simulink model "SolarPVMPPTBoost"  (R2025a)
settings: Solver=ode23t  StartTime=0.0  StopTime=simulation.timeSim  MaxStep=1/(10*solarPlant.converterSwitchingFrequency)  RelTol=1e-3  AbsTol=1e-3
PreLoadFcn:
  | run('SolarPVMPPTBoostData');
undefined symbols (not defined in the file or in its folder): boostController, dcVoltage, sensor, solarPanel, solarPlant
libraries: fl_lib x13, nesl_utility x9, simulink x6, ee_lib x3, eePwmGenerator x2, simulink_extras x1
Description:
  | Solar PV System with MPPT Using Boost Converter
  | 
  | %
settings Model: Creator=The MathWorks, Inc.  LastModifiedBy=The MathWorks, Inc.
settings SolverCC: AutoScaleAbsTol=off  AlgebraicLoopSolver=TrustRegion  MaxZcPerStep=1.0
settings DataIOCC: SaveOutput=off  DSMLogging=off  SaveTime=off  ReturnWorkspaceOutputs=off  SignalLoggingName=SolarPVMPPTBoost_logDB
settings OptimizationCC: ReuseModelBlockBuffer=off
settings DebuggingCC: UnconnectedInputMsg=warning  UnconnectedOutputMsg=warning  UnconnectedLineMsg=warning  SymbolicDimsDataTypeCodeGenerationDiagnostic=none
settings ModelReferenceCC: EnableRefExpFcnMdlSchedulingChecks=on
settings SFSimCC: CustomCodeUndefinedFunction=UseInterfaceOnly
settings RTWCC: GPUComputeCapability=3.5  DLArmComputeVersion=19.05
settings SimscapeCC: SimscapeLogType=all  SimscapeLogSimulationStatistics=on  SimscapeLogName=simlog_SolarPVMPPTBoost  SimscapeLogDataHistory=10000.0

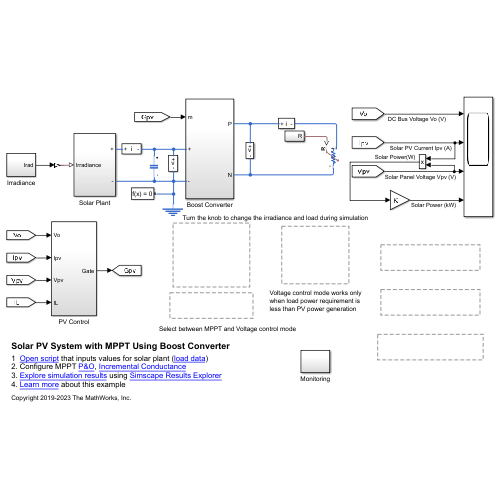
[thumbnail: Simulink's stored preview of the top-level diagram]
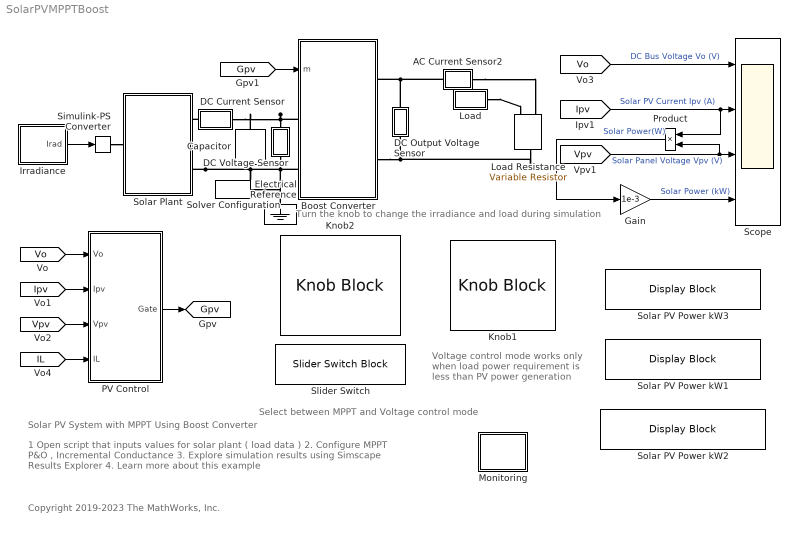
== system SolarPVMPPTBoost ==
  note: Turn the knob to change the irradiance and load during simulation
  note: Select between MPPT and Voltage control mode
  note: Voltage control mode works only when load power requirement is less than PV power generation
  note: Solar PV System with MPPT Using Boost Converter
  note: 1 Open script that inputs values for solar plant ( load data )
      | 2. Configure MPPT P&O , Incremental Conductance
      | 3. Explore simulation results using Simscape Results Explorer
      | 4. Learn more about this example
  note: Copyright 2019-2023 The MathWorks, Inc.
  AC Current Sensor2 : Subsystem
      mask Display: disp('i');
  Boost Converter : Subsystem  VariantControl=boostCircuit == 1
  Capacitor : fl_lib/Electrical/Electrical Elements/Capacitor  c=boost.inputCapacitor F  r=1e-6 Ohm  g=0 1/Ohm  i_specify=off  i_priority=None  i=0 A  i_nominal_specify=off  i_nominal_value=1  i_nominal_unit=A  v_specify=off  v_priority=None  v=solarPlant.startMPPTValue V  v_nominal_specify=off  v_nominal_value=1  v_nominal_unit=V  vc_specify=on  vc_priority=High  vc=solarPlant.startMPPTValue V  vc_nominal_specify=off  vc_nominal_value=1  vc_nominal_unit=V
  DC Current Sensor : Subsystem
      mask Display: disp('i')
  DC Output Voltage Sensor : Subsystem
      mask Display: disp('v')
  DC Voltage Sensor : Subsystem
      mask Display: disp('v');
  Electrical Reference : fl_lib/Electrical/Electrical Elements/Electrical Reference
  Gain : Gain  Gain=1e-3
  Irradiance : Subsystem
  Knob1 : KnobBlock  ScaleMin=0.1  ScaleMax=2  TickInterval=0.2
  Knob2 : KnobBlock  ScaleMin=150  ScaleMax=1000
  Load : Subsystem
  Load Resistance : fl_lib/Electrical/Electrical Elements/Variable Resistor  Rmin=0 Ohm  thermalEnable=false  thermal_mass=1 J/K  i_specify=off  i_priority=None  i=5 A  i_nominal_specify=off  i_nominal_value=1  i_nominal_unit=A  v_specify=off  v_priority=None  v=0 V  v_nominal_specify=off  v_nominal_value=1  v_nominal_unit=V  T_specify=off  T_priority=None  T=300 K  T_nominal_specify=off  T_nominal_value=1  T_nominal_unit=K
  Monitoring : Subsystem
  PV Control : Subsystem
  Product : Product
  Scope : Scope  NumInputPorts=4
      settings: TimeSpan=simulation.timeSim  ActiveDisplayYMinimum=-66.02811  ActiveDisplayYMaximum=594.25302
  Simulink-PS Converter : nesl_utility/Simulink-PS Converter  PhysicalDomain=network_engine_domain  SubClassName=ps_input  LeftPortType=input  RightPortType=output  PseudoPeriodic=off  Frequencies=[]  NoiseDistribution=none  NoiseParameters=[]  Unit=1  AffineConversion=off  FilteringAndDerivatives=provide  SimscapeFilterOrder=1  InputFilterTimeConstant=0.001  UdotUserProvided=0
  Slider Switch : SliderSwitchBlock
  Solar PV Power kW1 : DisplayBlock  Transparency=1  GridColor=[0.502, 0.502, 0.502]
  Solar PV Power kW2 : DisplayBlock  Transparency=1  GridColor=[0.502, 0.502, 0.502]
  Solar PV Power kW3 : DisplayBlock  Transparency=1  GridColor=[0.502, 0.502, 0.502]
  Solar Plant : Subsystem
  Solver Configuration : nesl_utility/Solver Configuration  PhysicalDomain=network_engine_domain  SubClassName=solver  LeftPortType=input  RightPortType=generic  Tones=[]  Harmonics=[]  SimulateNoise=off  Profile=off  UseLocalSampling=off  EnableSwitchedLinearOptims=on  FrequencyDomain=off  UseCCode=off  RelTol=0.001  AbsTol=1e-06  MinStep=1e-09  ToWorkspace=off  RevertToSquareIcSolve=off  NumHomotopyIterations=100  PhasorMode=off  PhasorModeNumHarmonics=1  ConsistencySolver=NEWTON_FTOL  IndexReductionMethod=DerivativeReplacement  DoDC=off  ResidualTolerance=1e-9  ConsistencyTolSource=GLOBAL  ConsistencyAbsTol=0.001  ConsistencyRelTol=0.001  ConsistencyTolFactor=0.001  UseLocalSolver=off  LocalSolverChoice=NE_BACKWARD_EULER_ADVANCER  ResolveIndetEquations=on  FunctionEvalNumThread=1  LocalSolverSampleTime=1e-6  DoFixedCost=off  MaxNonlinIter=10  MaxModeIter=2  ComputeImpulses=off  ImpulseIterations=2  LinearAlgebra=auto  LinearAlgebraNumThread=0  EquationFormulation=NE_TIME_EF  DelaysMemoryBudget=1024  AutomaticFiltering=on  FilteringTimeConstant=0.001  PartitionStorageMethod=AS_NEEDED  PartitionMemoryBudget=1024  PartitionMethod=FAST  MultibodyUseLocalSolver=off  MultibodyLocalSolverChoice=ODE1  MultibodyLocalSolverSampleTime=0.001
  tag scope: Gpv=global
  wires:
  PV Control/1(Gate) -> [Gpv]
  [Vo] -> Scope/1  "DC Bus Voltage Vo (V)"
  Irradiance/1(Irad) -> Simulink-PS Converter/1
  [Vpv] -> Product/2, Scope/3  "Solar Panel Voltage Vpv (V)"
  [Gpv] -> Boost Converter/1(m)
  [Vo] -> PV Control/1(Vo)
  [Ipv] -> Product/1, Scope/2  "Solar PV Current Ipv (A)"
  Product/1 -> Gain/1  "Solar Power(W)"
  Gain/1 -> Scope/4  "Solar Power (kW)"
  [Ipv] -> PV Control/2(Ipv)
  [Vpv] -> PV Control/3(Vpv)
  [IL] -> PV Control/4(IL)
  connections:
  Boost Converter/RConn2 -- Load Resistance/RConn1 -- DC Output Voltage Sensor/LConn1
  Solar Plant/RConn2 -- Solver Configuration/RConn1 -- Electrical Reference/LConn1 -- Boost Converter/LConn2 -- DC Voltage Sensor/LConn1 -- Capacitor/RConn1
  DC Voltage Sensor/RConn1 -- DC Current Sensor/LConn1 -- Capacitor/LConn1 -- Boost Converter/LConn1
  DC Output Voltage Sensor/RConn1 -- AC Current Sensor2/RConn1 -- Boost Converter/RConn1
  Simulink-PS Converter/RConn1 -- Solar Plant/LConn1
  DC Current Sensor/RConn1 -- Solar Plant/RConn1
  Load/RConn1 -- Load Resistance/LConn1
  AC Current Sensor2/LConn1 -- Load Resistance/LConn2

== system SolarPVMPPTBoost/AC Current Sensor2 ==
  Current Sensor : fl_lib/Electrical/Electrical Sensors/Current Sensor
  PS-Simulink Converter : nesl_utility/PS-Simulink Converter  PhysicalDomain=network_engine_domain  SubClassName=ps_output  LeftPortType=input  RightPortType=output  PseudoPeriodic=off  Frequencies=[]  VectorFormat=1-D array  Unit=1  AffineConversion=off
  Sensor dynamics : TransferFcn  Numerator=1  Denominator=[1/sensor.samplingFreq 1]
  - : PMIOPort  Side=Left
  + : PMIOPort  Port=2  Side=Right
  tag scope: Iload=global
  wires:
  PS-Simulink Converter/1 -> Sensor dynamics/1
  Sensor dynamics/1 -> [Iload]
  connections:
  Current Sensor/RConn1 -- PS-Simulink Converter/LConn1
  +/RConn1 -- Current Sensor/LConn1
  Current Sensor/RConn2 -- -/RConn1

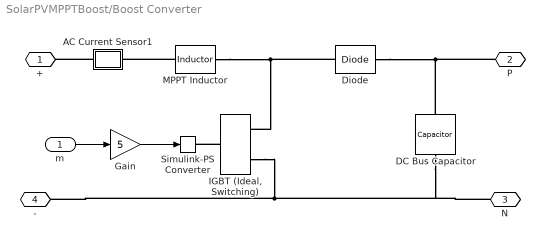
== system SolarPVMPPTBoost/Boost Converter ==
  m : Inport
  AC Current Sensor1 : Subsystem
      mask Display: disp('i');
  DC Bus Capacitor : fl_lib/Electrical/Electrical Elements/Capacitor  c=boost.outputCapacitor F  r=1e-6 Ohm  g=0 1/Ohm  i_specify=off  i_priority=None  i=0 A  i_nominal_specify=off  i_nominal_value=1  i_nominal_unit=A  v_specify=off  v_priority=None  v=0 V  v_nominal_specify=off  v_nominal_value=1  v_nominal_unit=V  vc_specify=on  vc_priority=High  vc=dcVoltage.avgDCVoltage V  vc_nominal_specify=off  vc_nominal_value=1  vc_nominal_unit=V
  Diode : fl_lib/Electrical/Electrical Elements/Diode  Vf=0.6 V  Ron=0.3 Ohm  Goff=1e-8 1/Ohm  i_specify=off  i_priority=None  i=0 A  i_nominal_specify=off  i_nominal_value=1  i_nominal_unit=A  v_specify=off  v_priority=None  v=0 V  v_nominal_specify=off  v_nominal_value=1  v_nominal_unit=V
  Gain : Gain  Gain=5
  "IGBT (Ideal, Switching)" : ee_lib/Semiconductors & Converters/IGBT (Ideal, Switching)  port_option=ee.enum.controlport.ps  Vf=0.8 V  Ron=0.001 Ohm  Goff=1e-5 1/Ohm  Vth=2.5 V  diode_param=1  diode_Vf=0.8 V  diode_Ron=0.001 Ohm  diode_Goff=1e-5 1/Ohm  diode_C=50e-9 F  diode_iRM=-235 A  diode_iF=300 A  diode_idot=-50 A/us  diode_trr_param=1  diode_trr_factor=3  diode_trr=15 us  diode_Qrr=1500 s*uA  ice_specify=off  ice_priority=None  ice=0 A  ice_nominal_specify=off  ice_nominal_value=1  ice_nominal_unit=A  vce_specify=off  vce_priority=None  vce=0 V  vce_nominal_specify=off  vce_nominal_value=1  vce_nominal_unit=V  vge_specify=off  vge_priority=None  vge=0 V  vge_nominal_specify=off  vge_nominal_value=1  vge_nominal_unit=V  thermal_loss_option=ee.enum.converters.thermalLossOption.constantvalues  Von_data=[0, .1, .6, .8, 1, 1.3, 1.6, 2, 2.4; 0, .1, .7, 1, 1.2, 1.5, 1.9, 2.4, 2.8] V  Tj=[298.15, 398.15] K  Iout_data=[0, .1, 1, 5, 10, 20, 40, 70, 100] A  Eon_data=[0, .0024, .024, .12, .2, .48, 1.04, 2.16, 3.24; 0, .003, .03, .15, .25, .6, 1.3, 2.7, 4.05] * 1e-3 J  Eoff_data=[0, .0007, .0066, .033, .066, .17, .33, .83, 1.5; 0, .001, .01, .05, .1, .25, .5, 1.2, 2.2] * 1e-3 J  Eon_data_3D=[zeros(2, 9, 3)] J  Eoff_data_3D=[zeros(2, 9, 3)] J  Tj_loss=[298.15, 398.15] K  Iout_data_loss=[0, .1, 1, 5, 10, 20, 40, 70, 100] A  tabulateWithVce=false  Vce_loss=[0, 150, 300] V  Eon_scalar=22.86e-3 J  Eoff_scalar=17.14e-3 J  Voff=300 V  Iout_scalar=600 A  useCurrentFromPreviousCycle=false  useVoltageFromPreviousCycle=false  diodeModelType=ee.enum.converters.diodeModelType.pwl  diodeTableType=ee.enum.diode.tableType.IfMat  diode_ReverseIVType=ee.enum.diode.diodeReverseIV.constant  diode_IfMat=[.07, .12, .19, 1.75, 4.24, 7.32, 11.2; .16, .3, .72, 2.14, 4.02, 6.35, 9.12] A  diode_VfMat=[.9, 1.15, 1.25, 1.5, 1.75, 2.17, 2.6, 2.85; .58, .68, .75, 1.1, 1.38, 1.77, 2.27, 2.7] V  diode_TjVec=[25, 125] degC  diode_VfVec=[.5, .7, .9, 1.3, 1.7, 2.1, 2.5] V  diode_IfVec=[.1, .2, .5, 1, 2, 4, 7, 10] A  diode_IrMat=[1e-06, 2e-06, 5e-06, 1e-05, 2.5e-05, 5e-05, .0001; 2e-06, 5e-06, 1e-05, 4e-05, 8e-05, .0002, .0005] A  diode_VrMat=[10, 100, 200, 250, 300, 325, 350; 10, 70, 160, 220, 270, 300, 320] V  diode_VrVec=[10, 20, 40, 50, 70, 80, 100] V  diode_IrVec=[1e-06, 2e-06, 5e-06, 1e-05, 2e-05, 5e-05, .0001] A  diode_Vr=-600 V  diode_Ls=150 nH  diode_Erec=0.03 J  diode_rec_loss_model=ee.enum.diode.reverseRecoveryModel.fixed  diode_ErecVal=0 J  diode_scaleWithIandV=true  diode_ErecMat=zeros(2, 3) J  diode_TjrecVec=[298.15, 398.15] K  diode_IfrecVec=[.1, 1, 10] A  diode_IrecVal=10 A  diode_VrecVal=10 V  diode_tFilter=1 / 1000 / 100 s  separateThermalPortForDiode=false  thermal_network_parameterization=ee.enum.thermalNetworkTopology.external  Rth=[.08, .5] K/W  Rth_Cauer=[.08, .1, .5] K/W  Rth_Foster=[.08, .14, .22, .16] K/W  thermal_mass_parameterization=ee.enum.thermalNetwork.timeconstant  thermal_mass=[.01, .5] J/K  thermal_mass_Cauer=[.01, .1, .5] J/K  thermal_mass_Foster=[.001, .005, .05, .5] J/K  thermal_time_constant=[.001, .2] s  thermal_time_constant_Cauer=[.001, .1, .2] s  thermal_time_constant_Foster=[7e-05, .0007, .01, .08] s  thermal_mass_initial_temperatures=[25, 25] degC  thermal_mass_initial_temperatures_Cauer=[25, 25, 25] degC  junction_thermal_mass=0.01 J/K  Tvec_initial_Foster=[25, 25, 25, 25] degC  RthDiode=[.03, .2] K/W  RthCauerDiode=[.03, .1, .2] K/W  RthFosterDiode=[.03, .2] K/W  thermalMassDiode=[3, 25] J/K  thermalMassCauerDiode=[3, 10, 25] J/K  thermalMassFosterDiode=[33, 50] J/K  thermalTauDiode=[.1, 5] s  thermalTauCauerDiode=[.1, 1, 5] s  thermalTauFosterDiode=[1, 10] s  thermalMassInitTempDiode=[25, 25] degC  thermalMassInitTempCauerDiode=[25, 25, 25] degC  junctionthermalMassDiode=0.1 J/K  TVecInitialFosterDiode=[25, 25, 25, 25] degC  no_thermal_network=0  IGBT_junction_temperature_specify=off  IGBT_junction_temperature_priority=None  IGBT_junction_temperature=25 degC  IGBT_junction_temperature_nominal_specify=off  IGBT_junction_temperature_nominal_value=1  IGBT_junction_temperature_nominal_unit=degC  diode_junction_temperature_specify=off  diode_junction_temperature_priority=None  diode_junction_temperature=25 degC  diode_junction_temperature_nominal_specify=off  diode_junction_temperature_nominal_value=1  diode_junction_temperature_nominal_unit=degC  Qj_specify=off  Qj_priority=None  Qj=0 W  Qj_nominal_specify=off  Qj_nominal_value=1  Qj_nominal_unit=W  accumulatedSwitchingLosses_specify=off  accumulatedSwitchingLosses_priority=None  accumulatedSwitchingLosses=0 J
  MPPT Inductor : ee_lib/Passive/Inductor  l=boost.inductor H  enable_L_tol=0  L_tol=5  tol_distribution=1  nSigma=4  r=boost.inductorResistance Ohm  g=1e-9 1/Ohm  enable_operating_limits=0  operating_limit_action=2  max_working_current=1 A  power_rating=1 W  i_L_specify=on  i_L_priority=High  i_L=0 A  i_L_nominal_specify=off  i_L_nominal_value=1  i_L_nominal_unit=A
  Simulink-PS Converter : nesl_utility/Simulink-PS Converter  PhysicalDomain=network_engine_domain  SubClassName=ps_input  LeftPortType=input  RightPortType=output  PseudoPeriodic=off  Frequencies=[]  NoiseDistribution=none  NoiseParameters=[]  Unit=1  AffineConversion=off  FilteringAndDerivatives=provide  SimscapeFilterOrder=1  InputFilterTimeConstant=0.001  UdotUserProvided=0
  + : PMIOPort  Side=Left
  P : PMIOPort  Port=2  Side=Right
  N : PMIOPort  Port=3  Side=Right
  - : PMIOPort  Port=4  Side=Left
  wires:
  m/1 -> Gain/1
  Gain/1 -> Simulink-PS Converter/1
  connections:
  MPPT Inductor/LConn1 -- AC Current Sensor1/LConn1
  "IGBT (Ideal, Switching)"/RConn2 -- N/RConn1 -- DC Bus Capacitor/RConn1 -- -/RConn1
  AC Current Sensor1/RConn1 -- +/RConn1
  "IGBT (Ideal, Switching)"/LConn1 -- Simulink-PS Converter/RConn1
  MPPT Inductor/RConn1 -- "IGBT (Ideal, Switching)"/RConn1 -- Diode/LConn1
  DC Bus Capacitor/LConn1 -- Diode/RConn1 -- P/RConn1

== system SolarPVMPPTBoost/DC Current Sensor ==
  Current Sensor : fl_lib/Electrical/Electrical Sensors/Current Sensor
      settings: LogSimulationData=on
  PS-Simulink Converter : nesl_utility/PS-Simulink Converter  PhysicalDomain=network_engine_domain  SubClassName=ps_output  LeftPortType=input  RightPortType=output  PseudoPeriodic=off  Frequencies=[]  VectorFormat=1-D array  Unit=1  AffineConversion=off
  Sensor dynamics : TransferFcn  Numerator=1  Denominator=[1/sensor.samplingFreq 1]
  - : PMIOPort  Side=Left
  + : PMIOPort  Port=2  Side=Right
  tag scope: Ipv=global
  wires:
  PS-Simulink Converter/1 -> Sensor dynamics/1
  Sensor dynamics/1 -> [Ipv]
  connections:
  Current Sensor/RConn2 -- -/RConn1
  +/RConn1 -- Current Sensor/LConn1
  Current Sensor/RConn1 -- PS-Simulink Converter/LConn1

== system SolarPVMPPTBoost/DC Output Voltage Sensor ==
  PS-Simulink Converter : nesl_utility/PS-Simulink Converter  PhysicalDomain=network_engine_domain  SubClassName=ps_output  LeftPortType=input  RightPortType=output  PseudoPeriodic=off  Frequencies=[]  VectorFormat=1-D array  Unit=1  AffineConversion=off
  Sensor dynamics : TransferFcn  Numerator=1  Denominator=[1/sensor.samplingFreq 1]
  Voltage Sensor : fl_lib/Electrical/Electrical Sensors/Voltage Sensor
  - : PMIOPort  Side=Left
  + : PMIOPort  Port=2  Side=Right
  tag scope: Vo=global
  wires:
  PS-Simulink Converter/1 -> Sensor dynamics/1
  Sensor dynamics/1 -> [Vo]
  connections:
  Voltage Sensor/RConn2 -- -/RConn1
  Voltage Sensor/RConn1 -- PS-Simulink Converter/LConn1
  Voltage Sensor/LConn1 -- +/RConn1

== system SolarPVMPPTBoost/DC Voltage Sensor ==
  PS-Simulink Converter : nesl_utility/PS-Simulink Converter  PhysicalDomain=network_engine_domain  SubClassName=ps_output  LeftPortType=input  RightPortType=output  PseudoPeriodic=off  Frequencies=[]  VectorFormat=1-D array  Unit=1  AffineConversion=off
  Sensor dynamics : TransferFcn  Numerator=1  Denominator=[1/sensor.samplingFreq 1]
  Voltage Sensor : fl_lib/Electrical/Electrical Sensors/Voltage Sensor
      settings: LogSimulationData=on
  - : PMIOPort  Side=Left
  + : PMIOPort  Port=2  Side=Right
  tag scope: Vpv=global
  wires:
  PS-Simulink Converter/1 -> Sensor dynamics/1
  Sensor dynamics/1 -> [Vpv]
  connections:
  Voltage Sensor/LConn1 -- +/RConn1
  Voltage Sensor/RConn1 -- PS-Simulink Converter/LConn1
  Voltage Sensor/RConn2 -- -/RConn1

== system SolarPVMPPTBoost/Irradiance ==
  " " : Constant
  Solar Irradiance W/m2 : Gain  Gain=988.0703074137369
  Irad : Outport
  wires:
  " "/1 -> Solar Irradiance W/m2/1
  Solar Irradiance W/m2/1 -> Irad/1

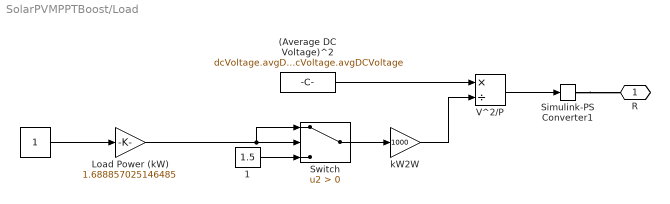
== system SolarPVMPPTBoost/Load ==
  " " : Constant
  " (Average DC Voltage)^2" : Constant  Value=dcVoltage.avgDCVoltage*dcVoltage.avgDCVoltage
  " 1" : Constant  Value=1.5
  Load Power (kW) : Gain  Gain=1.688857025146485
  Simulink-PS Converter1 : nesl_utility/Simulink-PS Converter  PhysicalDomain=network_engine_domain  SubClassName=ps_input  LeftPortType=input  RightPortType=output  PseudoPeriodic=off  Frequencies=[]  NoiseDistribution=none  NoiseParameters=[]  Unit=1  AffineConversion=off  FilteringAndDerivatives=provide  SimscapeFilterOrder=1  InputFilterTimeConstant=0.001  UdotUserProvided=0
  Switch : Switch  Criteria=u2 > Threshold  SaturateOnIntegerOverflow=off  InputSameDT=off
  V^2/P : Product  Inputs=*/
  kW2W : Gain  Gain=1000
  R : PMIOPort  Side=Right
  wires:
  " "/1 -> Load Power (kW)/1
  Load Power (kW)/1 -> Switch/1, Switch/2
  " 1"/1 -> Switch/3
  " (Average DC Voltage)^2"/1 -> V^2/P/1
  V^2/P/1 -> Simulink-PS Converter1/1
  Switch/1 -> kW2W/1
  kW2W/1 -> V^2/P/2
  connections:
  Simulink-PS Converter1/RConn1 -- R/RConn1

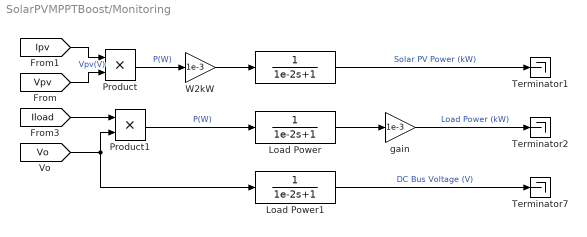
== system SolarPVMPPTBoost/Monitoring ==
  "  " : TransferFcn  Denominator=[1e-2 1]
  Load Power : TransferFcn  Denominator=[1e-2 1]
  Load Power1 : TransferFcn  Denominator=[1e-2 1]
  Product : Product
  Product1 : Product
  Terminator1 : Terminator
  Terminator2 : Terminator
  Terminator7 : Terminator
  W2kW : Gain  Gain=1e-3
  gain : Gain  Gain=1e-3
  wires:
  [Vpv] -> Product/2  "Vpv(V)"
  Load Power/1 -> gain/1
  Product1/1 -> Load Power/1  "P(W)"
  [Iload] -> Product1/1
  "  "/1 -> Terminator1/1  "Solar PV Power (kW)"
  [Ipv] -> Product/1
  [Vo] -> Product1/2, Load Power1/1
  Product/1 -> W2kW/1  "P(W)"
  gain/1 -> Terminator2/1  "Load Power (kW)"
  W2kW/1 -> "  "/1
  Load Power1/1 -> Terminator7/1  "DC Bus Voltage (V)"

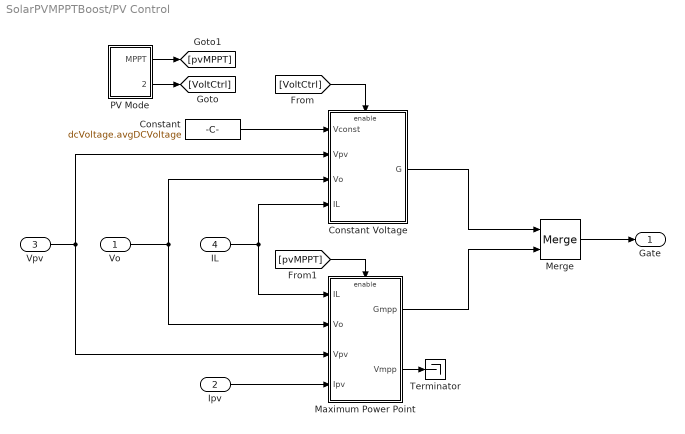
== system SolarPVMPPTBoost/PV Control ==
  Vo : Inport
  Ipv : Inport  Port=2
  Vpv : Inport  Port=3
  IL : Inport  Port=4
  Constant : Constant  Value=dcVoltage.avgDCVoltage
  Constant Voltage : Subsystem
  Maximum Power Point : Subsystem
  Merge : Merge
  PV Mode : Subsystem
  Terminator : Terminator
  Gate : Outport
  wires:
  Merge/1 -> Gate/1
  Vo/1 -> Maximum Power Point/2("Vo "), Constant Voltage/3("Vo ")
  Maximum Power Point/1(Gmpp) -> Merge/2
  [VoltCtrl] -> Constant Voltage/Enable
  IL/1 -> Maximum Power Point/1("IL "), Constant Voltage/4(IL)
  Vpv/1 -> Maximum Power Point/3(Vpv), Constant Voltage/2(Vpv)
  Ipv/1 -> Maximum Power Point/4(Ipv)
  Constant/1 -> Constant Voltage/1(Vconst)
  Constant Voltage/1(G) -> Merge/1
  Maximum Power Point/2(Vmpp) -> Terminator/1
  [pvMPPT] -> Maximum Power Point/Enable
  PV Mode/1(MPPT) -> [pvMPPT]
  PV Mode/2(VoltCtrl) -> [VoltCtrl]

== system SolarPVMPPTBoost/Solar Plant ==
  Current-Controlled Current Source- Scale panel current to Np parallel strings : fl_lib/Electrical/Electrical Sources/Current-Controlled Current Source  K=-1*(solarPlant.numParallelPanel-1)  i1_specify=off  i1_priority=None  i1=0 A  i1_nominal_specify=off  i1_nominal_value=1  i1_nominal_unit=A  i2_specify=off  i2_priority=None  i2=0 A  i2_nominal_specify=off  i2_nominal_value=1  i2_nominal_unit=A
      settings: InternalSimscapePortConfiguration="{\"Bottom\":[],\"Left\":[{\"id\":\"p1\",\"label\":\"+\",\"type\":\"foundation.electrical.electrical\"},{\"id\":\"head\",\"label\":\"\",\"type\":\"foundation.electrical.electrical\"}],\"Right\":[{\"id\":\"n1\",\"label\":\"-\",\"type\":\"foundation.electrical.electrical\"},{\"id\":\"tail\",\"label\":\"\",\"type\":\"foundation.electrical.electrical\"}],\"Top\":[]}"
  Solar Panel : Subsystem  mask(Solar Panel){}
      mask help: Models a solar panel using a parallel-connected sting of solar cells. The solar cell strings are modeled using a single Solar Cell block from the Simscape(TM) Electrical(TM) Sources library.
      mask Display: image('SolarPanelValidationIcon.jpg')
  Voltage-Controlled Voltage Source - Scale panel voltage to Ns series panel : fl_lib/Electrical/Electrical Sources/Voltage-Controlled Voltage Source  K=-1*(solarPlant.numSeriesPanel-1)  v1_specify=off  v1_priority=None  v1=0 V  v1_nominal_specify=off  v1_nominal_value=1  v1_nominal_unit=V  v2_specify=off  v2_priority=None  v2=0 V  v2_nominal_specify=off  v2_nominal_value=1  v2_nominal_unit=V
      settings: InternalSimscapePortConfiguration="{\"Bottom\":[],\"Left\":[{\"id\":\"p1\",\"label\":\"+\",\"type\":\"foundation.electrical.electrical\"},{\"id\":\"p2\",\"label\":\"+\",\"type\":\"foundation.electrical.electrical\"}],\"Right\":[{\"id\":\"n1\",\"label\":\"-\",\"type\":\"foundation.electrical.electrical\"},{\"id\":\"n2\",\"label\":\"-\",\"type\":\"foundation.electrical.electrical\"}],\"Top\":[]}"
  + : PMIOPort  Side=Right
  Irradiance : PMIOPort  Port=2  Side=Left
  - : PMIOPort  Port=3  Side=Right
  connections:
  Voltage-Controlled Voltage Source - Scale panel voltage to Ns series panel/RConn2 -- Voltage-Controlled Voltage Source - Scale panel voltage to Ns series panel/RConn1 -- Solar Panel/RConn1
  Voltage-Controlled Voltage Source - Scale panel voltage to Ns series panel/LConn1 -- Current-Controlled Current Source- Scale panel current to Np parallel strings/LConn2 -- -/RConn1 -- Solar Panel/RConn2
  Current-Controlled Current Source- Scale panel current to Np parallel strings/RConn1 -- Current-Controlled Current Source- Scale panel current to Np parallel strings/RConn2 -- +/RConn1
  Current-Controlled Current Source- Scale panel current to Np parallel strings/LConn1 -- Voltage-Controlled Voltage Source - Scale panel voltage to Ns series panel/LConn2
  Solar Panel/LConn1 -- Irradiance/RConn1

== system SolarPVMPPTBoost/Boost Converter/AC Current Sensor1 ==
  Current Sensor : fl_lib/Electrical/Electrical Sensors/Current Sensor
  PS-Simulink Converter : nesl_utility/PS-Simulink Converter  PhysicalDomain=network_engine_domain  SubClassName=ps_output  LeftPortType=input  RightPortType=output  PseudoPeriodic=off  Frequencies=[]  VectorFormat=1-D array  Unit=1  AffineConversion=off
  Sensor dynamics : TransferFcn  Numerator=1  Denominator=[1/sensor.samplingFreq 1]
  - : PMIOPort  Side=Left
  + : PMIOPort  Port=2  Side=Right
  tag scope: IL=global
  wires:
  PS-Simulink Converter/1 -> Sensor dynamics/1
  Sensor dynamics/1 -> [IL]
  connections:
  Current Sensor/RConn1 -- PS-Simulink Converter/LConn1
  +/RConn1 -- Current Sensor/LConn1
  Current Sensor/RConn2 -- -/RConn1

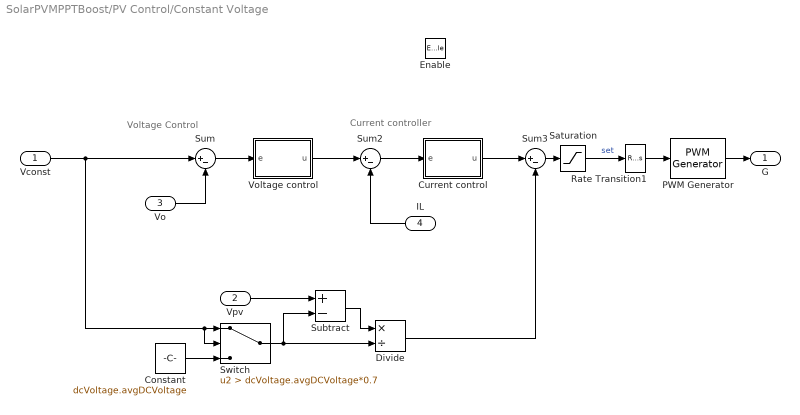
== system SolarPVMPPTBoost/PV Control/Constant Voltage ==
  note: Current controller
  note: Voltage Control
  Vconst : Inport
  Vpv : Inport  Port=2
  "Vo " : Inport  Port=3
  IL : Inport  Port=4
  Enable : EnablePort  StatesWhenEnabling=reset
  Constant : Constant  Value=dcVoltage.avgDCVoltage
  Current control : Subsystem
  Divide : Product  Inputs=*/
  PWM Generator : eePwmGenerator/PWM Generator  CarrCount=Up  Tper=1/solarPlant.converterSwitchingFrequency  Tdelay=0  Ts=1/(10*solarPlant.converterSwitchingFrequency)
  Rate Transition1 : RateTransition  OutPortSampleTime=1/(10*solarPlant.converterSwitchingFrequency)
  Saturation : Saturate  UpperLimit=1  LowerLimit=0
  Subtract : Sum  Inputs=+-
  Sum : Sum  Inputs=|+-
  Sum2 : Sum  Inputs=|+-
  Sum3 : Sum  Inputs=|+-
  Switch : Switch  Criteria=u2 > Threshold  Threshold=dcVoltage.avgDCVoltage*0.7  SaturateOnIntegerOverflow=off  InputSameDT=off
  Voltage control : Subsystem
  G : Outport
  wires:
  Switch/1 -> Divide/2, Subtract/2
  Constant/1 -> Switch/3
  "Vo "/1 -> Sum/2
  Vconst/1 -> Switch/2, Switch/1, Sum/1
  Divide/1 -> Sum3/2
  PWM Generator/1 -> G/1
  Rate Transition1/1 -> PWM Generator/1
  Sum3/1 -> Saturation/1
  Vpv/1 -> Subtract/1
  Sum/1 -> Voltage control/1(e)
  Voltage control/1(u) -> Sum2/1
  Current control/1(u) -> Sum3/1
  Sum2/1 -> Current control/1(e)
  Subtract/1 -> Divide/1
  Saturation/1 -> Rate Transition1/1  "set"
  IL/1 -> Sum2/2

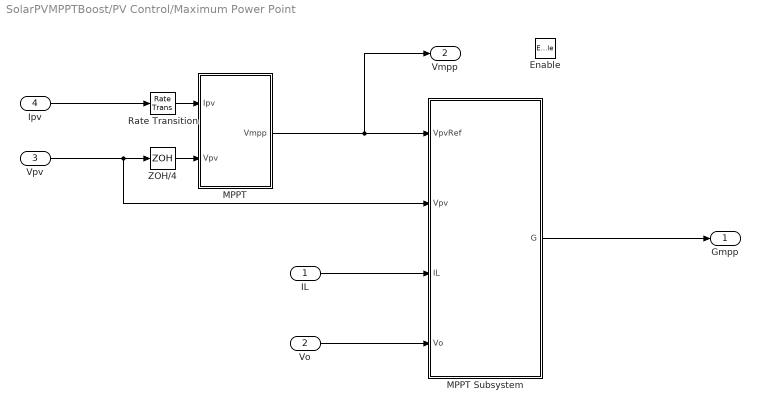
== system SolarPVMPPTBoost/PV Control/Maximum Power Point ==
  "IL " : Inport
  "Vo " : Inport  Port=2
  Vpv : Inport  Port=3
  Ipv : Inport  Port=4
  Enable : EnablePort  StatesWhenEnabling=reset
  MPPT : Subsystem
  MPPT Subsystem : Subsystem  TreatAsAtomicUnit=on
  Rate Transition : RateTransition  OutPortSampleTime=solarPlant.timeMPPT
  ZOH/4 : ZeroOrderHold  SampleTime=solarPlant.timeMPPT
  Gmpp : Outport
  Vmpp : Outport  Port=2
  wires:
  ZOH/4/1 -> MPPT/2(Vpv)
  Rate Transition/1 -> MPPT/1(Ipv)
  MPPT/1(Vmpp) -> Vmpp/1, MPPT Subsystem/1(VpvRef)
  "Vo "/1 -> MPPT Subsystem/4("Vo ")
  Ipv/1 -> Rate Transition/1
  Vpv/1 -> MPPT Subsystem/2(Vpv), ZOH/4/1
  MPPT Subsystem/1(G) -> Gmpp/1
  "IL "/1 -> MPPT Subsystem/3(IL)

== system SolarPVMPPTBoost/PV Control/PV Mode ==
  PV Mode : Constant
  PV Mode1 : Constant
  PV Mode2 : Constant  Value=0
  PV Mode3 : Constant
  Switch : Switch  Criteria=u2 > Threshold  Threshold=0.5  SaturateOnIntegerOverflow=off  InputSameDT=off
  Switch1 : Switch  Criteria=u2 > Threshold  Threshold=0.5  SaturateOnIntegerOverflow=off  InputSameDT=off
  MPPT : Outport
  VoltCtrl : Outport  Port=2
  wires:
  PV Mode1/1 -> Switch/1
  PV Mode/1 -> Switch/2, Switch1/2
  PV Mode2/1 -> Switch1/1, Switch/3
  Switch/1 -> MPPT/1
  PV Mode3/1 -> Switch1/3
  Switch1/1 -> VoltCtrl/1

== system SolarPVMPPTBoost/Solar Plant/Solar Panel ==
  Current-Controlled Current Source : fl_lib/Electrical/Electrical Sources/Current-Controlled Current Source  K=-1*(solarPanel.numParallelCell-1)  i1_specify=off  i1_priority=None  i1=0 A  i1_nominal_specify=off  i1_nominal_value=1  i1_nominal_unit=A  i2_specify=off  i2_priority=None  i2=0 A  i2_nominal_specify=off  i2_nominal_value=1  i2_nominal_unit=A
      settings: InternalSimscapePortConfiguration="{\"Bottom\":[],\"Left\":[{\"id\":\"p1\",\"label\":\"+\",\"type\":\"foundation.electrical.electrical\"},{\"id\":\"head\",\"label\":\"\",\"type\":\"foundation.electrical.electrical\"}],\"Right\":[{\"id\":\"n1\",\"label\":\"-\",\"type\":\"foundation.electrical.electrical\"},{\"id\":\"tail\",\"label\":\"\",\"type\":\"foundation.electrical.electrical\"}],\"Top\":[]}"
  Solar Cell : ee_lib/Sources/Solar Cell  prm=1  Isc=solarPanel.shortCircuitCurrentPV/solarPanel.numParallelCell A  Voc=solarPanel.openCircuitVoltagePV/solarPanel.numSeriesCell V  Is=1e-6 A  Is2=0 A  Iph=7.34 A  Ir0=solarPanel.irradianceMeasurement W/m^2  ec=solarPanel.qualityFactor  N2=2  Rs=solarPanel.seriesResistance Ohm  Rp=inf Ohm  N_series=solarPanel.numSeriesCell-1  N_parallel=1  TIPH1=solarPanel.currentTemperatureCoeff 1/K  EG=1.11 eV  TXIS1=solarPanel.temperatureExponent  TXIS2=3  TRS1=0  TRP1=0  Tmeas=solarPanel.temperatureMeasurement degC  TFIXED=environment.temperature degC  thermal_mass=100 J/K  initial_temperature=25 degC
  Ir : PMIOPort  Side=Left
  + : PMIOPort  Port=2  Side=Right
  - : PMIOPort  Port=3  Side=Right
  connections:
  Current-Controlled Current Source/LConn2 -- -/RConn1 -- Solar Cell/RConn1
  Ir/RConn1 -- Solar Cell/LConn1
  Current-Controlled Current Source/LConn1 -- Solar Cell/LConn2
  Current-Controlled Current Source/RConn1 -- Current-Controlled Current Source/RConn2 -- +/RConn1

== system SolarPVMPPTBoost/PV Control/Constant Voltage/Current control ==
  e : Inport
  Integrator : Integrator  LimitOutput=on  UpperSaturationLimit=1.5  LowerSaturationLimit=-1.5
  Ki : Gain  Gain=1/boostController.mppCurrentZeroTimeConst
  Kp : Gain  Gain=boostController.mppCurrentGain
  Saturation : Saturate  UpperLimit=1.5  LowerLimit=-1.5
  Sum7 : Sum  Inputs=|++
  u : Outport  VectorParamsAs1DForOutWhenUnconnected=off
  wires:
  Integrator/1 -> Sum7/2
  Saturation/1 -> u/1
  Sum7/1 -> Saturation/1
  e/1 -> Kp/1
  Kp/1 -> Ki/1, Sum7/1
  Ki/1 -> Integrator/1

== system SolarPVMPPTBoost/PV Control/Constant Voltage/Voltage control ==
  e : Inport
  1/T : Gain  Gain=1/boostController.mppVoltageZeroTimeConst
  Integrator : Integrator  LimitOutput=on  UpperSaturationLimit=boostController.mppVoltageLoopMax  LowerSaturationLimit=boostController.mppVoltageLoopMin
  Kp : Gain  Gain=boostController.mppVoltageGain
  Saturation : Saturate  UpperLimit=boostController.mppVoltageLoopMax  LowerLimit=boostController.mppVoltageLoopMin
  Sum7 : Sum  Inputs=|++
  u : Outport  VectorParamsAs1DForOutWhenUnconnected=off
  wires:
  Integrator/1 -> Sum7/2
  Saturation/1 -> u/1
  Sum7/1 -> Saturation/1
  e/1 -> Kp/1
  Kp/1 -> 1/T/1, Sum7/1
  1/T/1 -> Integrator/1

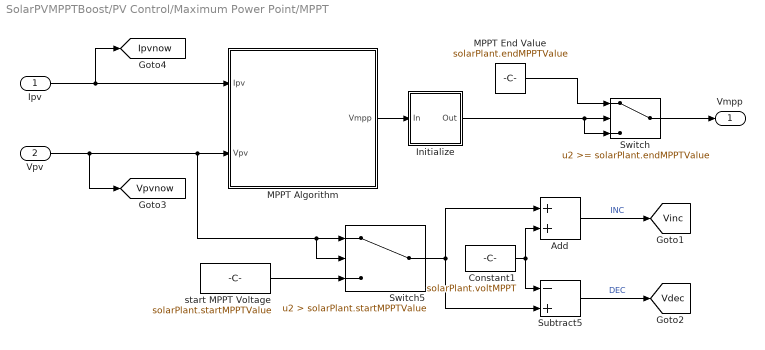
== system SolarPVMPPTBoost/PV Control/Maximum Power Point/MPPT ==
  Ipv : Inport
  Vpv : Inport  Port=2
  Add : Sum
  Constant1 : Constant  Value=solarPlant.voltMPPT
  Initialize : Subsystem
  MPPT Algorithm : Subsystem  Variant=on
  MPPT End Value : Constant  Value=solarPlant.endMPPTValue
  Subtract5 : Sum  Inputs=-+
  Switch : Switch  Threshold=solarPlant.endMPPTValue  SaturateOnIntegerOverflow=off  InputSameDT=off
  Switch5 : Switch  Criteria=u2 > Threshold  Threshold=solarPlant.startMPPTValue  SaturateOnIntegerOverflow=off  InputSameDT=off
  start MPPT Voltage : Constant  Value=solarPlant.startMPPTValue
  Vmpp : Outport  VectorParamsAs1DForOutWhenUnconnected=off
  tag scope: Ipvnow=global, Vdec=global, Vinc=global, Vpvnow=global
  wires:
  Switch5/1 -> Add/1, Subtract5/2
  Add/1 -> [Vinc]  "INC"
  start MPPT Voltage/1 -> Switch5/3
  Vpv/1 -> [Vpvnow], Switch5/2, Switch5/1, MPPT Algorithm/2(Vpv)
  Constant1/1 -> Add/2, Subtract5/1
  Subtract5/1 -> [Vdec]  "DEC"
  Ipv/1 -> [Ipvnow], MPPT Algorithm/1(Ipv)
  MPPT Algorithm/1(Vmpp) -> Initialize/1(In)
  Initialize/1(Out) -> Switch/3, Switch/2
  Switch/1 -> Vmpp/1
  MPPT End Value/1 -> Switch/1

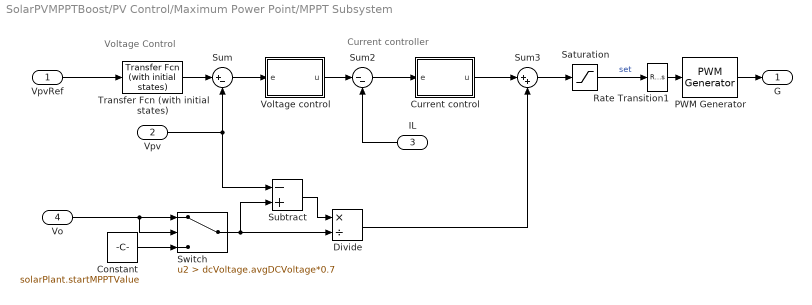
== system SolarPVMPPTBoost/PV Control/Maximum Power Point/MPPT Subsystem ==
  note: Current controller
  note: Voltage Control
  VpvRef : Inport
  Vpv : Inport  Port=2
  IL : Inport  Port=3
  "Vo " : Inport  Port=4
  Constant : Constant  Value=solarPlant.startMPPTValue
  Current control : Subsystem
  Divide : Product  Inputs=*/
  PWM Generator : eePwmGenerator/PWM Generator  CarrCount=Up  Tper=1/solarPlant.converterSwitchingFrequency  Tdelay=0  Ts=1/(10*solarPlant.converterSwitchingFrequency)
  Rate Transition1 : RateTransition  OutPortSampleTime=1/(10*solarPlant.converterSwitchingFrequency)
  Saturation : Saturate  UpperLimit=1  LowerLimit=0
  Subtract : Sum  Inputs=-+
  Sum : Sum  Inputs=|+-
  Sum2 : Sum  Inputs=|--
  Sum3 : Sum  Inputs=|++
  Switch : Switch  Criteria=u2 > Threshold  Threshold=dcVoltage.avgDCVoltage*0.7  SaturateOnIntegerOverflow=off  InputSameDT=off
  Transfer Fcn (with initial states) : simulink_extras/Additional Linear/Transfer Fcn (with initial states)  N=[1]  D=[0.00001 1]  X0=solarPlant.startMPPTValue
  Voltage control : Subsystem
  G : Outport
  wires:
  Subtract/1 -> Divide/1
  Voltage control/1(u) -> Sum2/1
  Current control/1(u) -> Sum3/1
  Sum2/1 -> Current control/1(e)
  "Vo "/1 -> Switch/2, Switch/1
  VpvRef/1 -> Transfer Fcn (with initial states)/1
  Constant/1 -> Switch/3
  Switch/1 -> Divide/2, Subtract/2
  Vpv/1 -> Subtract/1, Sum/2
  Saturation/1 -> Rate Transition1/1  "set"
  Rate Transition1/1 -> PWM Generator/1
  PWM Generator/1 -> G/1
  Divide/1 -> Sum3/2
  Sum/1 -> Voltage control/1(e)
  IL/1 -> Sum2/2
  Transfer Fcn (with initial states)/1 -> Sum/1
  Sum3/1 -> Saturation/1

== system SolarPVMPPTBoost/PV Control/Maximum Power Point/MPPT/Initialize ==
  In : Inport
  Constant : Constant  Value=solarPlant.startMPPTValue
  Constant2 : Constant
  Integrator : Integrator
  Switch1 : Switch  Criteria=u2 > Threshold  Threshold=solarPlant.startMPPTValue  SaturateOnIntegerOverflow=off  InputSameDT=off
  Switch2 : Switch  Criteria=u2 > Threshold  Threshold=solarPlant.timeMPPT  SaturateOnIntegerOverflow=off  InputSameDT=off
  Out : Outport
  wires:
  Constant/1 -> Switch1/3
  Switch1/1 -> Switch2/1
  In/1 -> Switch1/2, Switch1/1
  Switch2/1 -> Out/1
  Constant2/1 -> Integrator/1
  [Vpvnow] -> Switch2/3
  Integrator/1 -> Switch2/2

== system SolarPVMPPTBoost/PV Control/Maximum Power Point/MPPT/MPPT Algorithm ==
  Ipv : Inport
  Vpv : Inport  Port=2
  IncrementalConductance : Subsystem  VariantControl=incrementalConductance
  PerturbationAndObsrvation : Subsystem  VariantControl=perturbationAndObservation
  Vmpp : Outport  VectorParamsAs1DForOutWhenUnconnected=off

== system SolarPVMPPTBoost/PV Control/Maximum Power Point/MPPT Subsystem/Current control ==
  e : Inport
  Integrator : Integrator  InitialCondition=1  LimitOutput=on  UpperSaturationLimit=1  LowerSaturationLimit=-0.5
  Ki : Gain  Gain=1/boostController.mppCurrentZeroTimeConst
  Kp : Gain  Gain=boostController.mppCurrentGain
  Saturation : Saturate  UpperLimit=1  LowerLimit=-0.3
  Sum7 : Sum  Inputs=|++
  u : Outport  VectorParamsAs1DForOutWhenUnconnected=off
  wires:
  Integrator/1 -> Sum7/2
  Saturation/1 -> u/1
  Sum7/1 -> Saturation/1
  e/1 -> Kp/1
  Kp/1 -> Ki/1, Sum7/1
  Ki/1 -> Integrator/1

== system SolarPVMPPTBoost/PV Control/Maximum Power Point/MPPT Subsystem/Voltage control ==
  e : Inport
  1/T : Gain  Gain=1/boostController.mppVoltageZeroTimeConst
  Integrator : Integrator  LimitOutput=on  UpperSaturationLimit=boostController.mppVoltageLoopMax  LowerSaturationLimit=boostController.mppVoltageLoopMin
  Kp : Gain  Gain=boostController.mppVoltageGain
  Saturation : Saturate  UpperLimit=boostController.mppVoltageLoopMax  LowerLimit=boostController.mppVoltageLoopMin
  Sum7 : Sum  Inputs=|++
  u : Outport  VectorParamsAs1DForOutWhenUnconnected=off
  wires:
  Integrator/1 -> Sum7/2
  Saturation/1 -> u/1
  Sum7/1 -> Saturation/1
  e/1 -> Kp/1
  Kp/1 -> 1/T/1, Sum7/1
  1/T/1 -> Integrator/1

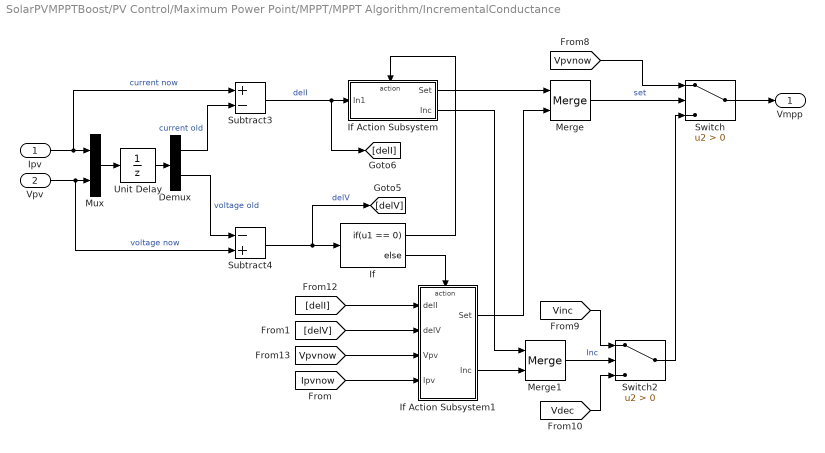
== system SolarPVMPPTBoost/PV Control/Maximum Power Point/MPPT/MPPT Algorithm/IncrementalConductance ==
  Ipv : Inport
  Vpv : Inport  Port=2
  Demux : Demux  Outputs=2
  If : If  IfExpression=u1 == 0
  If Action Subsystem : Subsystem  TreatAsAtomicUnit=on
  If Action Subsystem1 : Subsystem  TreatAsAtomicUnit=on
  Merge : Merge
  Merge1 : Merge
  Mux : Mux  Inputs=2
  Subtract3 : Sum  Inputs=+-
  Subtract4 : Sum  Inputs=-+
  Switch : Switch  Criteria=u2 > Threshold  SaturateOnIntegerOverflow=off  InputSameDT=off
  Switch2 : Switch  Criteria=u2 > Threshold  SaturateOnIntegerOverflow=off  InputSameDT=off
  Unit Delay : UnitDelay  InitialCondition=solarPlant.startMPPTValue  SampleTime=solarPlant.timeMPPT  HasFrameUpgradeWarning=on
  Vmpp : Outport  VectorParamsAs1DForOutWhenUnconnected=off
  wires:
  Merge1/1 -> Switch2/2  "Inc"
  [Vpvnow] -> Switch/1
  If Action Subsystem1/2(Inc) -> Merge1/2
  If Action Subsystem/2(Inc) -> Merge1/1
  If/2 -> If Action Subsystem1/Action
  If Action Subsystem/1(Set) -> Merge/1
  [delV] -> If Action Subsystem1/2(delV)
  [delI] -> If Action Subsystem1/1(delI)
  Merge/1 -> Switch/2  "set"
  If Action Subsystem1/1(Set) -> Merge/2
  If/1 -> If Action Subsystem/Action
  [Vpvnow] -> If Action Subsystem1/3(Vpv)
  Switch2/1 -> Switch/3
  [Ipvnow] -> If Action Subsystem1/4(Ipv)
  Ipv/1 -> Mux/1, Subtract3/1  "current now"
  Unit Delay/1 -> Demux/1
  Mux/1 -> Unit Delay/1
  Vpv/1 -> Subtract4/2, Mux/2  "voltage now"
  Demux/2 -> Subtract4/1  "voltage old"
  Demux/1 -> Subtract3/2  "current old"
  Subtract3/1 -> [delI], If Action Subsystem/1(In1)  "delI"
  Subtract4/1 -> [delV], If/1  "delV"
  Switch/1 -> Vmpp/1
  [Vdec] -> Switch2/3
  [Vinc] -> Switch2/1

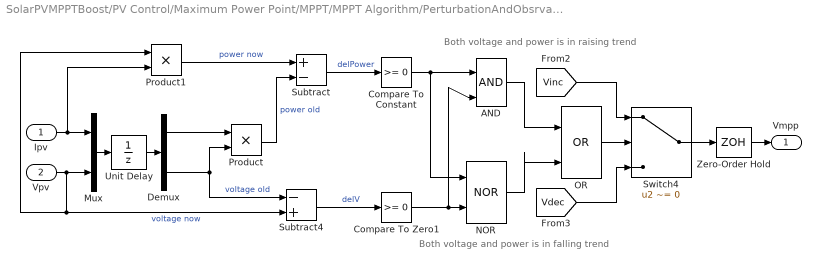
== system SolarPVMPPTBoost/PV Control/Maximum Power Point/MPPT/MPPT Algorithm/PerturbationAndObsrvation ==
  note: Both voltage and power is in falling trend
  note: Both voltage and power is in raising trend
  Ipv : Inport
  Vpv : Inport  Port=2
  AND : Logic  IconShape=distinctive  AllPortsSameDT=off  OutDataTypeStr=boolean
  Compare To Constant : simulink/Logic and Bit Operations/Compare To Constant  relop=>=  const=0  OutDataTypeStr=boolean
  Compare To Zero1 : simulink/Logic and Bit Operations/Compare To Zero  relop=>=  OutDataTypeStr=boolean
  Demux : Demux  Outputs=2
  Mux : Mux  Inputs=2
  NOR : Logic  Operator=NOR  IconShape=distinctive  AllPortsSameDT=off  OutDataTypeStr=boolean
  OR : Logic  Operator=OR  IconShape=distinctive  AllPortsSameDT=off  OutDataTypeStr=boolean
  Product : Product
  Product1 : Product
  Subtract : Sum  Inputs=+-
  Subtract4 : Sum  Inputs=-+
  Switch4 : Switch  Criteria=u2 ~= 0  SaturateOnIntegerOverflow=off  InputSameDT=off
  Unit Delay : UnitDelay  InitialCondition=solarPlant.startMPPTValue  SampleTime=solarPlant.timeMPPT  HasFrameUpgradeWarning=on
  Zero-Order Hold : ZeroOrderHold  SampleTime=solarPlant.timeMPPT
  Vmpp : Outport  VectorParamsAs1DForOutWhenUnconnected=off
  wires:
  NOR/1 -> OR/2
  OR/1 -> Switch4/2
  Compare To Zero1/1 -> AND/2, NOR/2
  AND/1 -> OR/1
  Compare To Constant/1 -> AND/1, NOR/1
  Mux/1 -> Unit Delay/1
  Ipv/1 -> Product1/2, Mux/1
  Demux/1 -> Product/1
  Unit Delay/1 -> Demux/1
  Demux/2 -> Product/2, Subtract4/1  "voltage old"
  Vpv/1 -> Product1/1, Subtract4/2, Mux/2  "voltage now"
  Product1/1 -> Subtract/1  "power now"
  Product/1 -> Subtract/2  "power old"
  Subtract4/1 -> Compare To Zero1/1  "delV"
  Subtract/1 -> Compare To Constant/1  "delPower"
  Switch4/1 -> Zero-Order Hold/1
  [Vdec] -> Switch4/3
  [Vinc] -> Switch4/1
  Zero-Order Hold/1 -> Vmpp/1

== system SolarPVMPPTBoost/PV Control/Maximum Power Point/MPPT/MPPT Algorithm/IncrementalConductance/If Action Subsystem ==
  In1 : Inport
  Action Port : ActionPort  ActionPortLabel=if(u1 == 0)
  Compare To Constant : simulink/Logic and Bit Operations/Compare To Constant  relop===  const=0  OutDataTypeStr=boolean
  Compare To Zero2 : simulink/Logic and Bit Operations/Compare To Zero  relop=>  OutDataTypeStr=boolean
  Set : Outport  VectorParamsAs1DForOutWhenUnconnected=off
  Inc : Outport  Port=2  VectorParamsAs1DForOutWhenUnconnected=off
  wires:
  Compare To Constant/1 -> Set/1  "Yes"
  Compare To Zero2/1 -> Inc/1  "Yes"
  In1/1 -> Compare To Zero2/1, Compare To Constant/1  "delI"

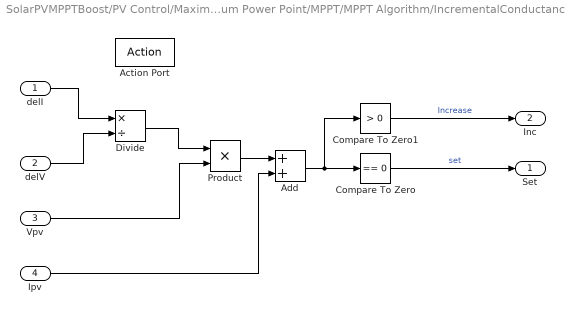
== system SolarPVMPPTBoost/PV Control/Maximum Power Point/MPPT/MPPT Algorithm/IncrementalConductance/If Action Subsystem1 ==
  delI : Inport
  delV : Inport  Port=2
  Vpv : Inport  Port=3
  Ipv : Inport  Port=4
  Action Port : ActionPort  ActionPortLabel=else
  Add : Sum
  Compare To Zero : simulink/Logic and Bit Operations/Compare To Zero  relop===  OutDataTypeStr=boolean
  Compare To Zero1 : simulink/Logic and Bit Operations/Compare To Zero  relop=>  OutDataTypeStr=boolean
  Divide : Product  Inputs=*/
  Product : Product
  Set : Outport  VectorParamsAs1DForOutWhenUnconnected=off
  Inc : Outport  Port=2  VectorParamsAs1DForOutWhenUnconnected=off
  wires:
  delI/1 -> Divide/1
  delV/1 -> Divide/2
  Divide/1 -> Product/1
  Add/1 -> Compare To Zero1/1, Compare To Zero/1
  Compare To Zero/1 -> Set/1  "set"
  Vpv/1 -> Product/2
  Product/1 -> Add/1
  Ipv/1 -> Add/2
  Compare To Zero1/1 -> Inc/1  "Increase"
